simulink model "SimulationPPU_Simscape"  (R2026a)
settings: Solver=ode23t  StopTime=10  MaxStep=1e-6  RelTol=1e-4
InitFcn:
  | % Read the SETTINGS constants on the top level
  | ppu_mdl = bdroot; ppu_mws = get_param(ppu_mdl, 'ModelWorkspace');
  | ppu_Fsw = slResolve(get_param([ppu_mdl '/Switching frequency'], 'Value'), ppu_mdl);
  | ppu_Vb  = slResolve(get_param([ppu_mdl '/DC bus voltage'], 'Value'), ppu_mdl);
  | assignin(ppu_mws, 'V_bus', ppu_Vb);            % initial DC-link voltage
  | set_param(ppu_mdl, 'MaxStep', sprintf('%.6g', 1/(20*ppu_Fsw)));
  | clear ppu_mdl ppu_mws ppu_Fsw ppu_Vb
model workspace (MAT data in the model file):
  C_cer = 3.36e-06
  C_elec = 0.0033
  C_f = 0.00088
  C_film = 4.5e-05
  ESR_cer = 0.0008
  ESR_elec = 0.023
  ESR_f = 0.057
  ESR_film = 0.0011
  Ki_I = 0.7
  Kp = 50
  Kp_I = 0.008
  L_Rser = 0.001
  L_f = 5.3e-05
  L_load = 0.0059
  N_par = 4
  R_Vsrc = 0.1
  R_load = 0.5
  Rb = 0.012
  Rd = 0.0092
  Rds_eq = 0.00440383953356
  Rg_ext = 1
  Rgs = 10000
  Ron_diode = 0.003
  Rs = 0.0069
  T_log = 2e-06
  T_stop = 0.2
  V_bus = 400
  Vf_diode = 0.65
  Vgs_on = 17.99820018
  Vhigh = 18
  Vto = 4.8
  m_max = 1.15470053838
  tau_Imeas = 0.001
libraries: fl_lib x23, nesl_utility x19, ee_lib x6, slpidlib x1, simulink x1
(part 1 of 2)
settings Model: SimulationMode=accelerator  Creator=gonzalo  LastModifiedBy=gonzalo
settings SolverCC: InitialStep=1e-9  MaxConsecutiveZCs=100000  MaxConsecutiveMinStep=100000  ZeroCrossAlgorithm=Adaptive
settings DebuggingCC: MaxConsecutiveZCsMsg=none  MaskedZcDiagnostic=none  IgnoredZcDiagnostic=none

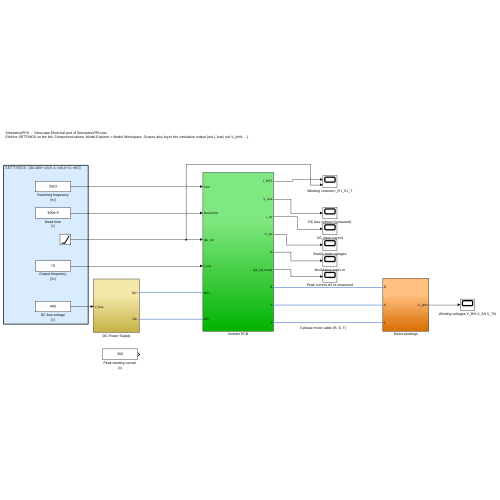
[thumbnail: Simulink's stored preview of the top-level diagram]
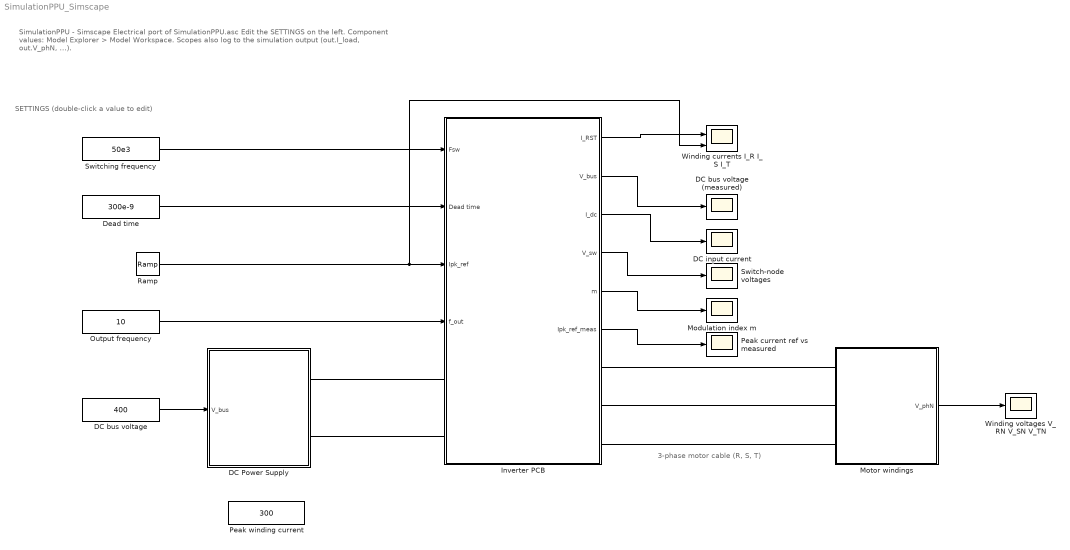
== system SimulationPPU_Simscape ==
  note: 3-phase motor cable (R, S, T)
  note: SETTINGS (double-click a value to edit)
  note: SimulationPPU  -  Simscape Electrical port of SimulationPPU.asc
      | Edit the SETTINGS on the left. Component values: Model Explorer > Model Workspace. Scopes also log to the simulation output (out.I_load, out.V_phN, ...).
  DC Power Supply : Subsystem
  DC bus voltage : Constant  Value=400
      settings: AttributesFormatString=[V]
  DC bus voltage (measured) : Scope
      settings: SampleTime=T_log  DataLoggingVariableName=V_bus_meas
  DC input current : Scope
      settings: SampleTime=T_log  DataLoggingVariableName=I_dc
  Dead time : Constant  Value=300e-9
      settings: AttributesFormatString=[s]
  Inverter PCB : Subsystem
  Modulation index m : Scope
      settings: SampleTime=T_log  DataLoggingVariableName=m
  Motor windings : Subsystem
  Output frequency : Constant  Value=10
      settings: AttributesFormatString=[Hz]
  Peak current ref vs measured : Scope
      settings: SampleTime=T_log  DataLoggingVariableName=Ipk_ref_meas
  Peak winding current : Constant  Value=300
      settings: AttributesFormatString=[A]
  Ramp : simulink/Sources/Ramp  slope=1  start=0  InitialOutput=10
  Switch-node voltages : Scope
      settings: SampleTime=T_log  DataLoggingVariableName=V_sw
  Switching frequency : Constant  Value=50e3
      settings: AttributesFormatString=[Hz]
  Winding currents I_R I_S I_T : Scope  NumInputPorts=2
      settings: SampleTime=T_log  DataLoggingVariableName=I_load
  Winding voltages V_RN V_SN V_TN : Scope
      settings: SampleTime=T_log  DataLoggingVariableName=V_phN
  wires:
  Switching frequency/1 -> Inverter PCB/1(Fsw)
  Dead time/1 -> Inverter PCB/2(Dead time)
  Ramp/1 -> Winding currents I_R I_S I_T/2, Inverter PCB/3(Ipk_ref)
  Output frequency/1 -> Inverter PCB/4(f_out)
  DC bus voltage/1 -> DC Power Supply/1(V_bus)
  Inverter PCB/1(I_RST) -> Winding currents I_R I_S I_T/1
  Inverter PCB/2(V_bus) -> DC bus voltage (measured)/1
  Inverter PCB/3(I_dc) -> DC input current/1
  Inverter PCB/4(V_sw) -> Switch-node voltages/1
  Inverter PCB/5(m) -> Modulation index m/1
  Inverter PCB/6(Ipk_ref_meas) -> Peak current ref vs measured/1
  Motor windings/1(V_phN) -> Winding voltages V_RN V_SN V_TN/1
  connections:
  DC Power Supply/RConn1 -- Inverter PCB/LConn1
  DC Power Supply/RConn2 -- Inverter PCB/LConn2
  Inverter PCB/RConn1 -- Motor windings/LConn1
  Inverter PCB/RConn2 -- Motor windings/LConn2
  Inverter PCB/RConn3 -- Motor windings/LConn3

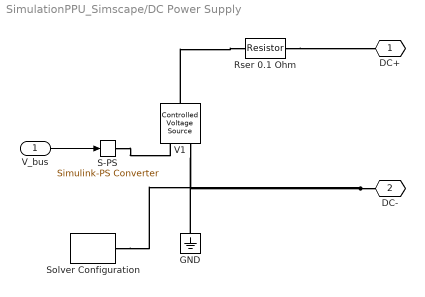
== system SimulationPPU_Simscape/DC Power Supply ==
  V_bus : Inport
  GND : fl_lib/Electrical/Electrical Elements/Electrical Reference
  Rser 0.1 Ohm : fl_lib/Electrical/Electrical Elements/Resistor  R=R_Vsrc Ohm  i_specify=off  i_priority=None  i=0 A  i_nominal_specify=off  i_nominal_value=1  i_nominal_unit=A  v_specify=off  v_priority=None  v=0 V  v_nominal_specify=off  v_nominal_value=1  v_nominal_unit=V
  S-PS : nesl_utility/Simulink-PS Converter  PhysicalDomain=network_engine_domain  SubClassName=ps_input  LeftPortType=input  RightPortType=output  PseudoPeriodic=off  Frequencies=[]  NoiseDistribution=none  NoiseParameters=[]  Unit=V  AffineConversion=off  FilteringAndDerivatives=zero  SimscapeFilterOrder=1  InputFilterTimeConstant=0.001  UdotUserProvided=0
  Solver Configuration : nesl_utility/Solver Configuration  PhysicalDomain=network_engine_domain  SubClassName=solver  LeftPortType=input  RightPortType=generic  Tones=[]  Harmonics=[]  SimulateNoise=off  Profile=off  UseLocalSampling=off  EnableSwitchedLinearOptims=on  FrequencyDomain=off  UseCCode=off  RelTol=0.001  AbsTol=0.001  MinStep=1e-09  ToWorkspace=off  RevertToSquareIcSolve=off  NumHomotopyIterations=100  PhasorMode=off  PhasorModeNumHarmonics=1  ConsistencySolver=NEWTON_XTOL_AFTER_FTOL  CanonicalOrdering=CANONICAL  OptimizeIntermediates=OPTIMIZED  IndexReductionMethod=DerivativeReplacement  DoDC=off  ResidualTolerance=1e-09  ConsistencyTolSource=GLOBAL  ConsistencyAbsTol=0.001  ConsistencyRelTol=0.001  ConsistencyTolFactor=0.001  UseLocalSolver=off  LocalSolverChoice=NE_BACKWARD_EULER_ADVANCER  ResolveIndetEquations=on  FunctionEvalNumThread=1  LocalSolverSampleTime=0.001  DoFixedCost=off  MaxNonlinIter=3  MaxModeIter=2  ComputeImpulses=off  ImpulseIterations=2  LinearAlgebra=auto  LinearAlgebraNumThread=0  EquationFormulation=NE_TIME_EF  DelaysMemoryBudget=1024  AutomaticFiltering=on  FilteringTimeConstant=0.001  PartitionStorageMethod=AS_NEEDED  PartitionMemoryBudget=1024  PartitionMethod=ROBUST  MultibodyUseLocalSolver=off  MultibodyLocalSolverChoice=ODE1  MultibodyLocalSolverSampleTime=0.001
  V1 : fl_lib/Electrical/Electrical Sources/Controlled Voltage Source
  DC+ : PMIOPort  Side=Right
  DC- : PMIOPort  Port=2  Side=Right
  wires:
  V_bus/1 -> S-PS/1
  connections:
  S-PS/RConn1 -- V1/RConn1
  V1/LConn1 -- Rser 0.1 Ohm/LConn1
  Rser 0.1 Ohm/RConn1 -- DC+/RConn1
  DC-/RConn1 -- V1/RConn2 -- GND/LConn1 -- Solver Configuration/RConn1

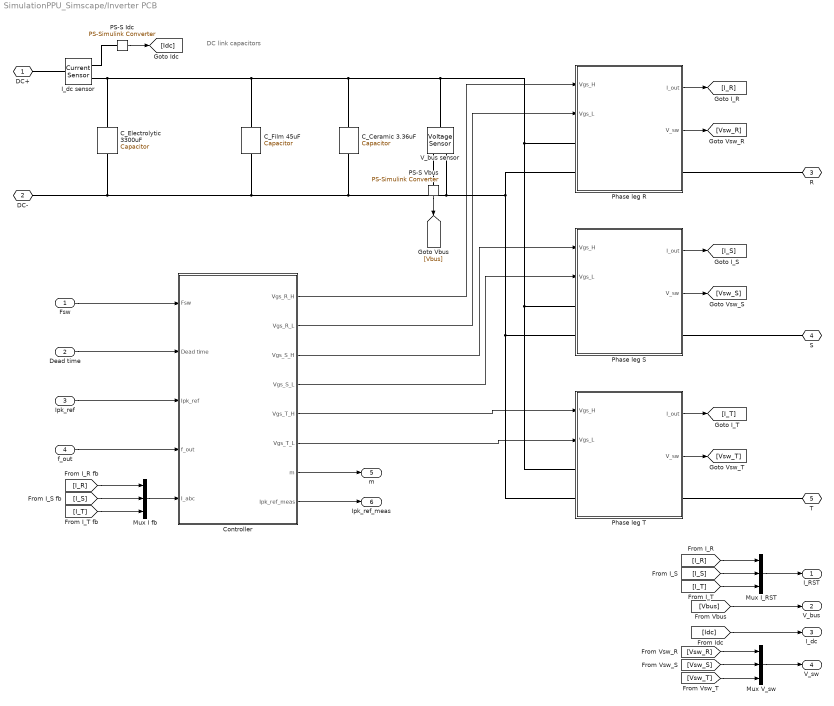
== system SimulationPPU_Simscape/Inverter PCB ==
  note: DC link capacitors
  Fsw : Inport
  Dead time : Inport  Port=2
  Ipk_ref : Inport  Port=3
  f_out : Inport  Port=4
  C_Ceramic 3.36uF : fl_lib/Electrical/Electrical Elements/Capacitor  c=C_cer F  r=ESR_cer Ohm  g=0 1/Ohm  i_specify=off  i_priority=None  i=0 A  i_nominal_specify=off  i_nominal_value=1  i_nominal_unit=A  v_specify=off  v_priority=None  v=0 V  v_nominal_specify=off  v_nominal_value=1  v_nominal_unit=V  vc_specify=on  vc_priority=High  vc=V_bus V  vc_nominal_specify=off  vc_nominal_value=1  vc_nominal_unit=V
  C_Electrolytic 3300uF : fl_lib/Electrical/Electrical Elements/Capacitor  c=C_elec F  r=ESR_elec Ohm  g=0 1/Ohm  i_specify=off  i_priority=None  i=0 A  i_nominal_specify=off  i_nominal_value=1  i_nominal_unit=A  v_specify=off  v_priority=None  v=0 V  v_nominal_specify=off  v_nominal_value=1  v_nominal_unit=V  vc_specify=on  vc_priority=High  vc=V_bus V  vc_nominal_specify=off  vc_nominal_value=1  vc_nominal_unit=V
  C_Film 45uF : fl_lib/Electrical/Electrical Elements/Capacitor  c=C_film F  r=ESR_film Ohm  g=0 1/Ohm  i_specify=off  i_priority=None  i=0 A  i_nominal_specify=off  i_nominal_value=1  i_nominal_unit=A  v_specify=off  v_priority=None  v=0 V  v_nominal_specify=off  v_nominal_value=1  v_nominal_unit=V  vc_specify=on  vc_priority=High  vc=V_bus V  vc_nominal_specify=off  vc_nominal_value=1  vc_nominal_unit=V
  Controller : Subsystem
  I_dc sensor : fl_lib/Electrical/Electrical Sensors/Current Sensor
  Mux I fb : Mux  Inputs=3
  Mux I_RST : Mux  Inputs=3
  Mux V_sw : Mux  Inputs=3
  PS-S Idc : nesl_utility/PS-Simulink Converter  PhysicalDomain=network_engine_domain  SubClassName=ps_output  LeftPortType=input  RightPortType=output  PseudoPeriodic=off  Frequencies=[]  VectorFormat=inherit  Unit=inherit  AffineConversion=off
  PS-S Vbus : nesl_utility/PS-Simulink Converter  PhysicalDomain=network_engine_domain  SubClassName=ps_output  LeftPortType=input  RightPortType=output  PseudoPeriodic=off  Frequencies=[]  VectorFormat=inherit  Unit=inherit  AffineConversion=off
  Phase leg R : Subsystem
  Phase leg S : Subsystem
  Phase leg T : Subsystem
  V_bus sensor : fl_lib/Electrical/Electrical Sensors/Voltage Sensor
  DC+ : PMIOPort  Side=Left
  DC- : PMIOPort  Port=2  Side=Left
  R : PMIOPort  Port=3  Side=Right
  S : PMIOPort  Port=4  Side=Right
  T : PMIOPort  Port=5  Side=Right
  I_RST : Outport
  V_bus : Outport  Port=2
  I_dc : Outport  Port=3
  V_sw : Outport  Port=4
  m : Outport  Port=5
  Ipk_ref_meas : Outport  Port=6
  wires:
  PS-S Idc/1 -> [Idc]
  PS-S Vbus/1 -> [Vbus]
  Phase leg R/1(I_out) -> [I_R]
  Phase leg R/2(V_sw) -> [Vsw_R]
  Phase leg S/1(I_out) -> [I_S]
  Phase leg S/2(V_sw) -> [Vsw_S]
  Phase leg T/1(I_out) -> [I_T]
  Phase leg T/2(V_sw) -> [Vsw_T]
  Fsw/1 -> Controller/1(Fsw)
  Dead time/1 -> Controller/2(Dead time)
  Ipk_ref/1 -> Controller/3(Ipk_ref)
  f_out/1 -> Controller/4(f_out)
  Mux I fb/1 -> Controller/5(I_abc)
  [I_R] -> Mux I fb/1
  [I_S] -> Mux I fb/2
  [I_T] -> Mux I fb/3
  Controller/1(Vgs_R_H) -> Phase leg R/1(Vgs_H)
  Controller/2(Vgs_R_L) -> Phase leg R/2(Vgs_L)
  Controller/3(Vgs_S_H) -> Phase leg S/1(Vgs_H)
  Controller/4(Vgs_S_L) -> Phase leg S/2(Vgs_L)
  Controller/5(Vgs_T_H) -> Phase leg T/1(Vgs_H)
  Controller/6(Vgs_T_L) -> Phase leg T/2(Vgs_L)
  Mux I_RST/1 -> I_RST/1
  [I_R] -> Mux I_RST/1
  [I_S] -> Mux I_RST/2
  [I_T] -> Mux I_RST/3
  Mux V_sw/1 -> V_sw/1
  [Vsw_R] -> Mux V_sw/1
  [Vsw_S] -> Mux V_sw/2
  [Vsw_T] -> Mux V_sw/3
  [Vbus] -> V_bus/1
  [Idc] -> I_dc/1
  Controller/7(m) -> m/1
  Controller/8(Ipk_ref_meas) -> Ipk_ref_meas/1
  connections:
  DC+/RConn1 -- I_dc sensor/LConn1
  I_dc sensor/RConn1 -- PS-S Idc/LConn1
  I_dc sensor/RConn2 -- C_Electrolytic 3300uF/LConn1 -- C_Film 45uF/LConn1 -- C_Ceramic 3.36uF/LConn1 -- V_bus sensor/LConn1 -- Phase leg R/LConn1 -- Phase leg S/LConn1 -- Phase leg T/LConn1
  DC-/RConn1 -- C_Electrolytic 3300uF/RConn1 -- C_Film 45uF/RConn1 -- C_Ceramic 3.36uF/RConn1 -- V_bus sensor/RConn2 -- Phase leg R/LConn2 -- Phase leg S/LConn2 -- Phase leg T/LConn2
  V_bus sensor/RConn1 -- PS-S Vbus/LConn1
  Phase leg R/RConn1 -- R/RConn1
  Phase leg S/RConn1 -- S/RConn1
  Phase leg T/RConn1 -- T/RConn1

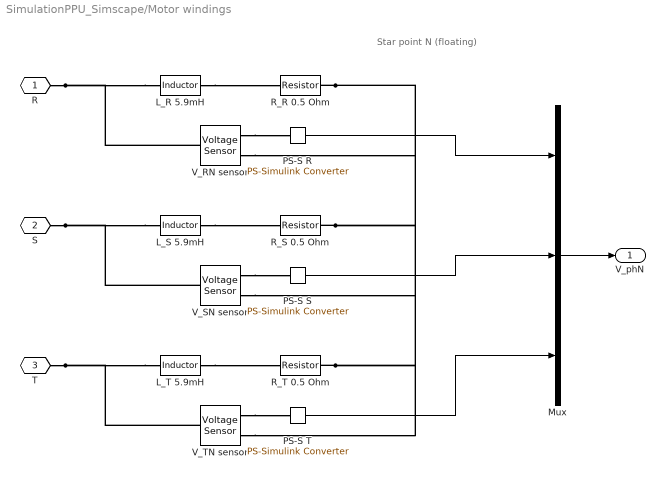
== system SimulationPPU_Simscape/Motor windings ==
  note: Star point N (floating)
  L_R 5.9mH : fl_lib/Electrical/Electrical Elements/Inductor  l=L_load H  r=L_Rser Ohm  g=0 1/Ohm  i_specify=off  i_priority=None  i=0 A  i_nominal_specify=off  i_nominal_value=1  i_nominal_unit=A  v_specify=off  v_priority=None  v=0 V  v_nominal_specify=off  v_nominal_value=1  v_nominal_unit=V  i_L_specify=off  i_L_priority=High  i_L=0 A  i_L_nominal_specify=off  i_L_nominal_value=1  i_L_nominal_unit=A
  L_S 5.9mH : fl_lib/Electrical/Electrical Elements/Inductor  l=L_load H  r=L_Rser Ohm  g=0 1/Ohm  i_specify=off  i_priority=None  i=0 A  i_nominal_specify=off  i_nominal_value=1  i_nominal_unit=A  v_specify=off  v_priority=None  v=0 V  v_nominal_specify=off  v_nominal_value=1  v_nominal_unit=V  i_L_specify=off  i_L_priority=High  i_L=0 A  i_L_nominal_specify=off  i_L_nominal_value=1  i_L_nominal_unit=A
  L_T 5.9mH : fl_lib/Electrical/Electrical Elements/Inductor  l=L_load H  r=L_Rser Ohm  g=0 1/Ohm  i_specify=off  i_priority=None  i=0 A  i_nominal_specify=off  i_nominal_value=1  i_nominal_unit=A  v_specify=off  v_priority=None  v=0 V  v_nominal_specify=off  v_nominal_value=1  v_nominal_unit=V  i_L_specify=off  i_L_priority=High  i_L=0 A  i_L_nominal_specify=off  i_L_nominal_value=1  i_L_nominal_unit=A
  Mux : Mux  Inputs=3
  PS-S R : nesl_utility/PS-Simulink Converter  PhysicalDomain=network_engine_domain  SubClassName=ps_output  LeftPortType=input  RightPortType=output  PseudoPeriodic=off  Frequencies=[]  VectorFormat=inherit  Unit=inherit  AffineConversion=off
  PS-S S : nesl_utility/PS-Simulink Converter  PhysicalDomain=network_engine_domain  SubClassName=ps_output  LeftPortType=input  RightPortType=output  PseudoPeriodic=off  Frequencies=[]  VectorFormat=inherit  Unit=inherit  AffineConversion=off
  PS-S T : nesl_utility/PS-Simulink Converter  PhysicalDomain=network_engine_domain  SubClassName=ps_output  LeftPortType=input  RightPortType=output  PseudoPeriodic=off  Frequencies=[]  VectorFormat=inherit  Unit=inherit  AffineConversion=off
  R_R 0.5 Ohm : fl_lib/Electrical/Electrical Elements/Resistor  R=R_load Ohm  i_specify=off  i_priority=None  i=0 A  i_nominal_specify=off  i_nominal_value=1  i_nominal_unit=A  v_specify=off  v_priority=None  v=0 V  v_nominal_specify=off  v_nominal_value=1  v_nominal_unit=V
  R_S 0.5 Ohm : fl_lib/Electrical/Electrical Elements/Resistor  R=R_load Ohm  i_specify=off  i_priority=None  i=0 A  i_nominal_specify=off  i_nominal_value=1  i_nominal_unit=A  v_specify=off  v_priority=None  v=0 V  v_nominal_specify=off  v_nominal_value=1  v_nominal_unit=V
  R_T 0.5 Ohm : fl_lib/Electrical/Electrical Elements/Resistor  R=R_load Ohm  i_specify=off  i_priority=None  i=0 A  i_nominal_specify=off  i_nominal_value=1  i_nominal_unit=A  v_specify=off  v_priority=None  v=0 V  v_nominal_specify=off  v_nominal_value=1  v_nominal_unit=V
  V_RN sensor : fl_lib/Electrical/Electrical Sensors/Voltage Sensor
  V_SN sensor : fl_lib/Electrical/Electrical Sensors/Voltage Sensor
  V_TN sensor : fl_lib/Electrical/Electrical Sensors/Voltage Sensor
  R : PMIOPort  Side=Left
  S : PMIOPort  Port=2  Side=Left
  T : PMIOPort  Port=3  Side=Left
  V_phN : Outport
  wires:
  Mux/1 -> V_phN/1
  PS-S R/1 -> Mux/1
  PS-S S/1 -> Mux/2
  PS-S T/1 -> Mux/3
  connections:
  L_R 5.9mH/LConn1 -- R/RConn1 -- V_RN sensor/LConn1
  L_R 5.9mH/RConn1 -- R_R 0.5 Ohm/LConn1
  R_R 0.5 Ohm/RConn1 -- V_RN sensor/RConn2 -- V_SN sensor/RConn2 -- R_S 0.5 Ohm/RConn1 -- V_TN sensor/RConn2 -- R_T 0.5 Ohm/RConn1
  V_RN sensor/RConn1 -- PS-S R/LConn1
  L_S 5.9mH/LConn1 -- S/RConn1 -- V_SN sensor/LConn1
  L_S 5.9mH/RConn1 -- R_S 0.5 Ohm/LConn1
  V_SN sensor/RConn1 -- PS-S S/LConn1
  L_T 5.9mH/LConn1 -- T/RConn1 -- V_TN sensor/LConn1
  L_T 5.9mH/RConn1 -- R_T 0.5 Ohm/LConn1
  V_TN sensor/RConn1 -- PS-S T/LConn1

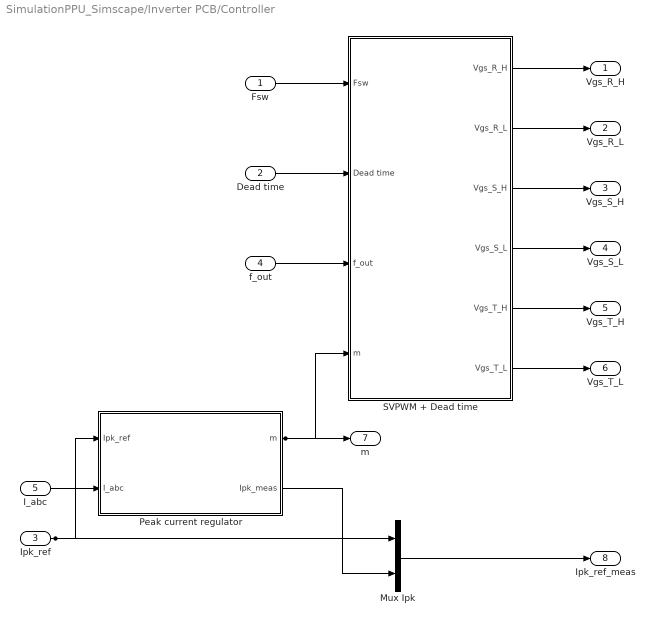
== system SimulationPPU_Simscape/Inverter PCB/Controller ==
  Fsw : Inport
  Dead time : Inport  Port=2
  Ipk_ref : Inport  Port=3
  f_out : Inport  Port=4
  I_abc : Inport  Port=5
  Mux Ipk : Mux  Inputs=2
  Peak current regulator : Subsystem
  SVPWM + Dead time : Subsystem
  Vgs_R_H : Outport
  Vgs_R_L : Outport  Port=2
  Vgs_S_H : Outport  Port=3
  Vgs_S_L : Outport  Port=4
  Vgs_T_H : Outport  Port=5
  Vgs_T_L : Outport  Port=6
  m : Outport  Port=7
  Ipk_ref_meas : Outport  Port=8
  wires:
  Mux Ipk/1 -> Ipk_ref_meas/1
  I_abc/1 -> Peak current regulator/2(I_abc)
  Peak current regulator/1(m) -> m/1, SVPWM + Dead time/4(m)
  Ipk_ref/1 -> Peak current regulator/1(Ipk_ref), Mux Ipk/1
  SVPWM + Dead time/5(Vgs_T_H) -> Vgs_T_H/1
  Fsw/1 -> SVPWM + Dead time/1(Fsw)
  SVPWM + Dead time/4(Vgs_S_L) -> Vgs_S_L/1
  Dead time/1 -> SVPWM + Dead time/2(Dead time)
  SVPWM + Dead time/2(Vgs_R_L) -> Vgs_R_L/1
  f_out/1 -> SVPWM + Dead time/3(f_out)
  SVPWM + Dead time/1(Vgs_R_H) -> Vgs_R_H/1
  Peak current regulator/2(Ipk_meas) -> Mux Ipk/2
  SVPWM + Dead time/6(Vgs_T_L) -> Vgs_T_L/1
  SVPWM + Dead time/3(Vgs_S_H) -> Vgs_S_H/1

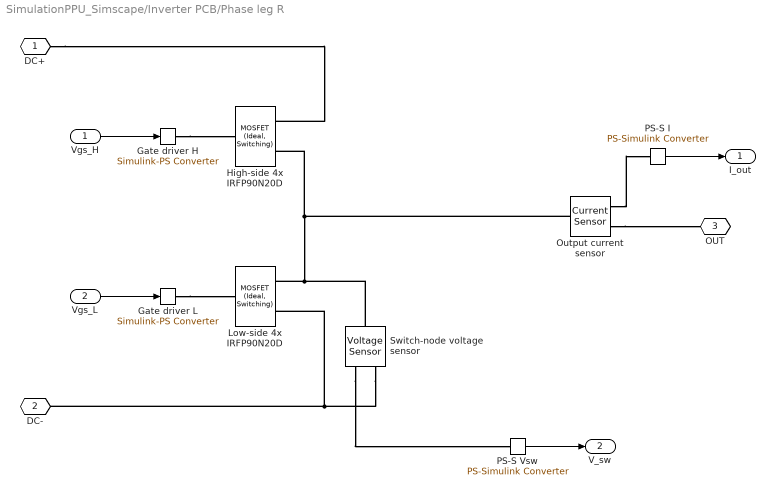
== system SimulationPPU_Simscape/Inverter PCB/Phase leg R ==
  Vgs_H : Inport
  Vgs_L : Inport  Port=2
  Gate driver H : nesl_utility/Simulink-PS Converter  PhysicalDomain=network_engine_domain  SubClassName=ps_input  LeftPortType=input  RightPortType=output  PseudoPeriodic=off  Frequencies=[]  NoiseDistribution=none  NoiseParameters=[]  Unit=V  AffineConversion=off  FilteringAndDerivatives=zero  SimscapeFilterOrder=1  InputFilterTimeConstant=0.001  UdotUserProvided=0
  Gate driver L : nesl_utility/Simulink-PS Converter  PhysicalDomain=network_engine_domain  SubClassName=ps_input  LeftPortType=input  RightPortType=output  PseudoPeriodic=off  Frequencies=[]  NoiseDistribution=none  NoiseParameters=[]  Unit=V  AffineConversion=off  FilteringAndDerivatives=zero  SimscapeFilterOrder=1  InputFilterTimeConstant=0.001  UdotUserProvided=0
  High-side 4x IRFP90N20D : ee_lib/Semiconductors & Converters/MOSFET (Ideal, Switching)  port_option=ee.enum.controlport.ps  Rds=Rds_eq Ohm  Goff=1e-7 1/Ohm  Vth=Vto V  diode_param=ee.enum.semiconductors.protectionDiode.nodynamics  diode_Vf=Vf_diode V  diode_Ron=Ron_diode Ohm  diode_Goff=1e-7 1/Ohm  diode_C=50e-9 F  diode_iRM=-235 A  diode_iF=300 A  diode_idot=-50 A/us  diode_trr_param=ee.enum.converters.diodeReverseParam.trr_factor  diode_trr_factor=3  diode_trr=15 us  diode_Qrr=1500 s*uA  ids_specify=off  ids_priority=None  ids=0 A  ids_nominal_specify=off  ids_nominal_value=1  ids_nominal_unit=A  vds_specify=off  vds_priority=None  vds=0 V  vds_nominal_specify=off  vds_nominal_value=1  vds_nominal_unit=V  vgs_specify=off  vgs_priority=None  vgs=0 V  vgs_nominal_specify=off  vgs_nominal_value=1  vgs_nominal_unit=V  thermal_loss_option=ee.enum.converters.thermalLossOption.constantvalues  Von_data=[0, 1.8, 3.2, 6, 10, 16; 0, 2, 5.5, 9.5, 15, 25] V  Tj=[298.15, 448.15] K  Iout_data=[0, 20, 40, 60, 80, 100] A  tabulateWithVds=false  Eon_data=[0, 55.04, 124.57, 235.53, 362.12; 0, 71.25, 161.25, 304.88, 468.75] * 1e-6 J  Eoff_data=[0, 18, 30, 56.1, 76.5; 0, 22.5, 37.5, 70.13, 95.63] * 1e-6 J  Eon_data_3D=[zeros(2, 5, 3)] J  Eoff_data_3D=[zeros(2, 5, 3)] J  Tj_loss=[298.15, 448.15] K  Iout_data_loss=[0, 10, 20, 30, 40] A  Vds_loss=[0, 150, 300] V  Eon_scalar=22.86e-3 J  Eoff_scalar=17.14e-3 J  Voff=300 V  Iout_scalar=600 A  useCurrentFromPreviousCycle=false  useVoltageFromPreviousCycle=false  diodeModelType=ee.enum.converters.diodeModelType.pwl  diodeTableType=ee.enum.diode.tableType.IfMat  diode_ReverseIVType=ee.enum.diode.diodeReverseIV.constant  diode_IfMat=[.07, .12, .19, 1.75, 4.24, 7.32, 11.2; .16, .3, .72, 2.14, 4.02, 6.35, 9.12] A  diode_VfMat=[.9, 1.15, 1.25, 1.5, 1.75, 2.17, 2.6, 2.85; .58, .68, .75, 1.1, 1.38, 1.77, 2.27, 2.7] V  diode_TjVec=[25, 125] degC  diode_VfVec=[.5, .7, .9, 1.3, 1.7, 2.1, 2.5] V  diode_IfVec=[.1, .2, .5, 1, 2, 4, 7, 10] A  diode_IrMat=[1e-06, 2e-06, 5e-06, 1e-05, 2.5e-05, 5e-05, .0001; 2e-06, 5e-06, 1e-05, 4e-05, 8e-05, .0002, .0005] A  diode_VrMat=[10, 100, 200, 250, 300, 325, 350; 10, 70, 160, 220, 270, 300, 320] V  diode_VrVec=[10, 20, 40, 50, 70, 80, 100] V  diode_IrVec=[1e-06, 2e-06, 5e-06, 1e-05, 2e-05, 5e-05, .0001] A  diode_Vr=-600 V  diode_Ls=150 nH  diode_Erec=0.03 J  diode_rec_loss_model=ee.enum.diode.reverseRecoveryModelTabulateUpTo3D.fixed  diode_ErecVal=0 J  diode_scaleWithIandV=true  diode_ErecMat=zeros(2, 3) J  diodeErecMat3D=zeros(2, 3, 2) J  diode_TjrecVec=[298.15, 398.15] K  diode_IfrecVec=[.1, 1, 10] A  diodeVrecVec=[0, 100] V  diode_IrecVal=10 A  diode_VrecVal=10 V  diode_tFilter=1 / 1000 / 100 s  separateThermalPortForDiode=false  thermal_network_parameterization=ee.enum.thermalNetworkTopology.external  Rth=[.03, .2] K/W  Rth_Cauer=[.03, .1, .2] K/W  Rth_Foster=[.08, .14, .22, .16] K/W  thermal_mass_parameterization=ee.enum.thermalNetwork.timeconstant  thermal_mass=[3, 25] J/K  thermal_mass_Cauer=[3, 10, 25] J/K  thermal_mass_Foster=[.001, .005, .05, .5] J/K  thermal_time_constant=[.1, 5] s  thermal_time_constant_Cauer=[.1, 1, 5] s  thermal_time_constant_Foster=[7e-05, .0007, .01, .08] s  thermal_mass_initial_temperatures=[25, 25] degC  thermal_mass_initial_temperatures_Cauer=[25, 25, 25] degC  junction_thermal_mass=0.1 J/K  Tvec_initial_Foster=[25, 25, 25, 25] degC  RthDiode=[.03, .2] K/W  RthCauerDiode=[.03, .1, .2] K/W  RthFosterDiode=[.03, .2] K/W  thermalMassDiode=[3, 25] J/K  thermalMassCauerDiode=[3, 10, 25] J/K  thermalMassFosterDiode=[33, 50] J/K  thermalTauDiode=[.1, 5] s  thermalTauCauerDiode=[.1, 1, 5] s  thermalTauFosterDiode=[1, 10] s  thermalMassInitTempDiode=[25, 25] degC  thermalMassInitTempCauerDiode=[25, 25, 25] degC  junctionthermalMassDiode=0.1 J/K  TVecInitialFosterDiode=[25, 25, 25, 25] degC  no_thermal_network=ee.enum.enable.no  mosfet_junction_temperature_specify=off  mosfet_junction_temperature_priority=None  mosfet_junction_temperature=25 degC  mosfet_junction_temperature_nominal_specify=off  mosfet_junction_temperature_nominal_value=1  mosfet_junction_temperature_nominal_unit=degC  diode_junction_temperature_specify=off  diode_junction_temperature_priority=None  diode_junction_temperature=25 degC  diode_junction_temperature_nominal_specify=off  diode_junction_temperature_nominal_value=1  diode_junction_temperature_nominal_unit=degC  Qj_specify=off  Qj_priority=None  Qj=0 W  Qj_nominal_specify=off  Qj_nominal_value=1  Qj_nominal_unit=W  accumulatedSwitchingLosses_specify=off  accumulatedSwitchingLosses_priority=None  accumulatedSwitchingLosses=0 J
  Low-side 4x IRFP90N20D : ee_lib/Semiconductors & Converters/MOSFET (Ideal, Switching)  port_option=ee.enum.controlport.ps  Rds=Rds_eq Ohm  Goff=1e-7 1/Ohm  Vth=Vto V  diode_param=ee.enum.semiconductors.protectionDiode.nodynamics  diode_Vf=Vf_diode V  diode_Ron=Ron_diode Ohm  diode_Goff=1e-7 1/Ohm  diode_C=50e-9 F  diode_iRM=-235 A  diode_iF=300 A  diode_idot=-50 A/us  diode_trr_param=ee.enum.converters.diodeReverseParam.trr_factor  diode_trr_factor=3  diode_trr=15 us  diode_Qrr=1500 s*uA  ids_specify=off  ids_priority=None  ids=0 A  ids_nominal_specify=off  ids_nominal_value=1  ids_nominal_unit=A  vds_specify=off  vds_priority=None  vds=0 V  vds_nominal_specify=off  vds_nominal_value=1  vds_nominal_unit=V  vgs_specify=off  vgs_priority=None  vgs=0 V  vgs_nominal_specify=off  vgs_nominal_value=1  vgs_nominal_unit=V  thermal_loss_option=ee.enum.converters.thermalLossOption.constantvalues  Von_data=[0, 1.8, 3.2, 6, 10, 16; 0, 2, 5.5, 9.5, 15, 25] V  Tj=[298.15, 448.15] K  Iout_data=[0, 20, 40, 60, 80, 100] A  tabulateWithVds=false  Eon_data=[0, 55.04, 124.57, 235.53, 362.12; 0, 71.25, 161.25, 304.88, 468.75] * 1e-6 J  Eoff_data=[0, 18, 30, 56.1, 76.5; 0, 22.5, 37.5, 70.13, 95.63] * 1e-6 J  Eon_data_3D=[zeros(2, 5, 3)] J  Eoff_data_3D=[zeros(2, 5, 3)] J  Tj_loss=[298.15, 448.15] K  Iout_data_loss=[0, 10, 20, 30, 40] A  Vds_loss=[0, 150, 300] V  Eon_scalar=22.86e-3 J  Eoff_scalar=17.14e-3 J  Voff=300 V  Iout_scalar=600 A  useCurrentFromPreviousCycle=false  useVoltageFromPreviousCycle=false  diodeModelType=ee.enum.converters.diodeModelType.pwl  diodeTableType=ee.enum.diode.tableType.IfMat  diode_ReverseIVType=ee.enum.diode.diodeReverseIV.constant  diode_IfMat=[.07, .12, .19, 1.75, 4.24, 7.32, 11.2; .16, .3, .72, 2.14, 4.02, 6.35, 9.12] A  diode_VfMat=[.9, 1.15, 1.25, 1.5, 1.75, 2.17, 2.6, 2.85; .58, .68, .75, 1.1, 1.38, 1.77, 2.27, 2.7] V  diode_TjVec=[25, 125] degC  diode_VfVec=[.5, .7, .9, 1.3, 1.7, 2.1, 2.5] V  diode_IfVec=[.1, .2, .5, 1, 2, 4, 7, 10] A  diode_IrMat=[1e-06, 2e-06, 5e-06, 1e-05, 2.5e-05, 5e-05, .0001; 2e-06, 5e-06, 1e-05, 4e-05, 8e-05, .0002, .0005] A  diode_VrMat=[10, 100, 200, 250, 300, 325, 350; 10, 70, 160, 220, 270, 300, 320] V  diode_VrVec=[10, 20, 40, 50, 70, 80, 100] V  diode_IrVec=[1e-06, 2e-06, 5e-06, 1e-05, 2e-05, 5e-05, .0001] A  diode_Vr=-600 V  diode_Ls=150 nH  diode_Erec=0.03 J  diode_rec_loss_model=ee.enum.diode.reverseRecoveryModelTabulateUpTo3D.fixed  diode_ErecVal=0 J  diode_scaleWithIandV=true  diode_ErecMat=zeros(2, 3) J  diodeErecMat3D=zeros(2, 3, 2) J  diode_TjrecVec=[298.15, 398.15] K  diode_IfrecVec=[.1, 1, 10] A  diodeVrecVec=[0, 100] V  diode_IrecVal=10 A  diode_VrecVal=10 V  diode_tFilter=1 / 1000 / 100 s  separateThermalPortForDiode=false  thermal_network_parameterization=ee.enum.thermalNetworkTopology.external  Rth=[.03, .2] K/W  Rth_Cauer=[.03, .1, .2] K/W  Rth_Foster=[.08, .14, .22, .16] K/W  thermal_mass_parameterization=ee.enum.thermalNetwork.timeconstant  thermal_mass=[3, 25] J/K  thermal_mass_Cauer=[3, 10, 25] J/K  thermal_mass_Foster=[.001, .005, .05, .5] J/K  thermal_time_constant=[.1, 5] s  thermal_time_constant_Cauer=[.1, 1, 5] s  thermal_time_constant_Foster=[7e-05, .0007, .01, .08] s  thermal_mass_initial_temperatures=[25, 25] degC  thermal_mass_initial_temperatures_Cauer=[25, 25, 25] degC  junction_thermal_mass=0.1 J/K  Tvec_initial_Foster=[25, 25, 25, 25] degC  RthDiode=[.03, .2] K/W  RthCauerDiode=[.03, .1, .2] K/W  RthFosterDiode=[.03, .2] K/W  thermalMassDiode=[3, 25] J/K  thermalMassCauerDiode=[3, 10, 25] J/K  thermalMassFosterDiode=[33, 50] J/K  thermalTauDiode=[.1, 5] s  thermalTauCauerDiode=[.1, 1, 5] s  thermalTauFosterDiode=[1, 10] s  thermalMassInitTempDiode=[25, 25] degC  thermalMassInitTempCauerDiode=[25, 25, 25] degC  junctionthermalMassDiode=0.1 J/K  TVecInitialFosterDiode=[25, 25, 25, 25] degC  no_thermal_network=ee.enum.enable.no  mosfet_junction_temperature_specify=off  mosfet_junction_temperature_priority=None  mosfet_junction_temperature=25 degC  mosfet_junction_temperature_nominal_specify=off  mosfet_junction_temperature_nominal_value=1  mosfet_junction_temperature_nominal_unit=degC  diode_junction_temperature_specify=off  diode_junction_temperature_priority=None  diode_junction_temperature=25 degC  diode_junction_temperature_nominal_specify=off  diode_junction_temperature_nominal_value=1  diode_junction_temperature_nominal_unit=degC  Qj_specify=off  Qj_priority=None  Qj=0 W  Qj_nominal_specify=off  Qj_nominal_value=1  Qj_nominal_unit=W  accumulatedSwitchingLosses_specify=off  accumulatedSwitchingLosses_priority=None  accumulatedSwitchingLosses=0 J
  Output current sensor : fl_lib/Electrical/Electrical Sensors/Current Sensor
  PS-S I : nesl_utility/PS-Simulink Converter  PhysicalDomain=network_engine_domain  SubClassName=ps_output  LeftPortType=input  RightPortType=output  PseudoPeriodic=off  Frequencies=[]  VectorFormat=inherit  Unit=inherit  AffineConversion=off
  PS-S Vsw : nesl_utility/PS-Simulink Converter  PhysicalDomain=network_engine_domain  SubClassName=ps_output  LeftPortType=input  RightPortType=output  PseudoPeriodic=off  Frequencies=[]  VectorFormat=inherit  Unit=inherit  AffineConversion=off
  Switch-node voltage sensor : fl_lib/Electrical/Electrical Sensors/Voltage Sensor
  DC+ : PMIOPort  Side=Left
  DC- : PMIOPort  Port=2  Side=Left
  OUT : PMIOPort  Port=3  Side=Right
  I_out : Outport
  V_sw : Outport  Port=2
  wires:
  Vgs_H/1 -> Gate driver H/1
  Vgs_L/1 -> Gate driver L/1
  PS-S I/1 -> I_out/1
  PS-S Vsw/1 -> V_sw/1
  connections:
  Gate driver H/RConn1 -- High-side 4x IRFP90N20D/LConn1
  Gate driver L/RConn1 -- Low-side 4x IRFP90N20D/LConn1
  DC+/RConn1 -- High-side 4x IRFP90N20D/RConn1
  Output current sensor/LConn1 -- High-side 4x IRFP90N20D/RConn2 -- Low-side 4x IRFP90N20D/RConn1 -- Switch-node voltage sensor/LConn1
  DC-/RConn1 -- Switch-node voltage sensor/RConn2 -- Low-side 4x IRFP90N20D/RConn2
  Output current sensor/RConn2 -- OUT/RConn1
  Output current sensor/RConn1 -- PS-S I/LConn1
  Switch-node voltage sensor/RConn1 -- PS-S Vsw/LConn1

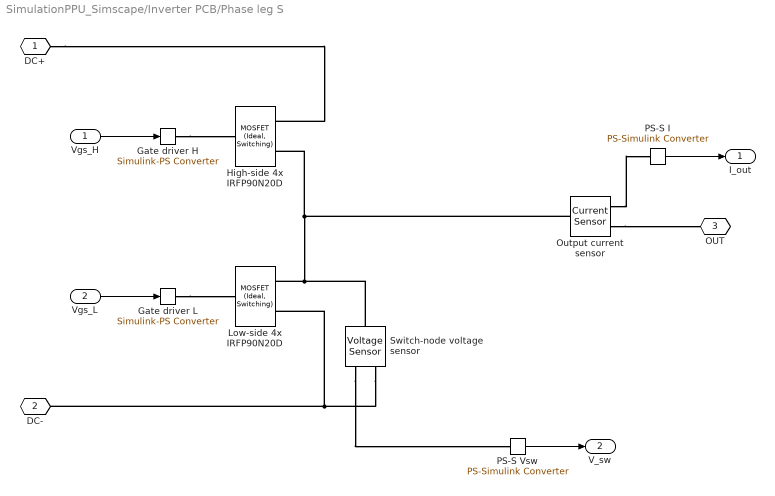
== system SimulationPPU_Simscape/Inverter PCB/Phase leg S ==
  Vgs_H : Inport
  Vgs_L : Inport  Port=2
  Gate driver H : nesl_utility/Simulink-PS Converter  PhysicalDomain=network_engine_domain  SubClassName=ps_input  LeftPortType=input  RightPortType=output  PseudoPeriodic=off  Frequencies=[]  NoiseDistribution=none  NoiseParameters=[]  Unit=V  AffineConversion=off  FilteringAndDerivatives=zero  SimscapeFilterOrder=1  InputFilterTimeConstant=0.001  UdotUserProvided=0
  Gate driver L : nesl_utility/Simulink-PS Converter  PhysicalDomain=network_engine_domain  SubClassName=ps_input  LeftPortType=input  RightPortType=output  PseudoPeriodic=off  Frequencies=[]  NoiseDistribution=none  NoiseParameters=[]  Unit=V  AffineConversion=off  FilteringAndDerivatives=zero  SimscapeFilterOrder=1  InputFilterTimeConstant=0.001  UdotUserProvided=0
  High-side 4x IRFP90N20D : ee_lib/Semiconductors & Converters/MOSFET (Ideal, Switching)  port_option=ee.enum.controlport.ps  Rds=Rds_eq Ohm  Goff=1e-7 1/Ohm  Vth=Vto V  diode_param=ee.enum.semiconductors.protectionDiode.nodynamics  diode_Vf=Vf_diode V  diode_Ron=Ron_diode Ohm  diode_Goff=1e-7 1/Ohm  diode_C=50e-9 F  diode_iRM=-235 A  diode_iF=300 A  diode_idot=-50 A/us  diode_trr_param=ee.enum.converters.diodeReverseParam.trr_factor  diode_trr_factor=3  diode_trr=15 us  diode_Qrr=1500 s*uA  ids_specify=off  ids_priority=None  ids=0 A  ids_nominal_specify=off  ids_nominal_value=1  ids_nominal_unit=A  vds_specify=off  vds_priority=None  vds=0 V  vds_nominal_specify=off  vds_nominal_value=1  vds_nominal_unit=V  vgs_specify=off  vgs_priority=None  vgs=0 V  vgs_nominal_specify=off  vgs_nominal_value=1  vgs_nominal_unit=V  thermal_loss_option=ee.enum.converters.thermalLossOption.constantvalues  Von_data=[0, 1.8, 3.2, 6, 10, 16; 0, 2, 5.5, 9.5, 15, 25] V  Tj=[298.15, 448.15] K  Iout_data=[0, 20, 40, 60, 80, 100] A  tabulateWithVds=false  Eon_data=[0, 55.04, 124.57, 235.53, 362.12; 0, 71.25, 161.25, 304.88, 468.75] * 1e-6 J  Eoff_data=[0, 18, 30, 56.1, 76.5; 0, 22.5, 37.5, 70.13, 95.63] * 1e-6 J  Eon_data_3D=[zeros(2, 5, 3)] J  Eoff_data_3D=[zeros(2, 5, 3)] J  Tj_loss=[298.15, 448.15] K  Iout_data_loss=[0, 10, 20, 30, 40] A  Vds_loss=[0, 150, 300] V  Eon_scalar=22.86e-3 J  Eoff_scalar=17.14e-3 J  Voff=300 V  Iout_scalar=600 A  useCurrentFromPreviousCycle=false  useVoltageFromPreviousCycle=false  diodeModelType=ee.enum.converters.diodeModelType.pwl  diodeTableType=ee.enum.diode.tableType.IfMat  diode_ReverseIVType=ee.enum.diode.diodeReverseIV.constant  diode_IfMat=[.07, .12, .19, 1.75, 4.24, 7.32, 11.2; .16, .3, .72, 2.14, 4.02, 6.35, 9.12] A  diode_VfMat=[.9, 1.15, 1.25, 1.5, 1.75, 2.17, 2.6, 2.85; .58, .68, .75, 1.1, 1.38, 1.77, 2.27, 2.7] V  diode_TjVec=[25, 125] degC  diode_VfVec=[.5, .7, .9, 1.3, 1.7, 2.1, 2.5] V  diode_IfVec=[.1, .2, .5, 1, 2, 4, 7, 10] A  diode_IrMat=[1e-06, 2e-06, 5e-06, 1e-05, 2.5e-05, 5e-05, .0001; 2e-06, 5e-06, 1e-05, 4e-05, 8e-05, .0002, .0005] A  diode_VrMat=[10, 100, 200, 250, 300, 325, 350; 10, 70, 160, 220, 270, 300, 320] V  diode_VrVec=[10, 20, 40, 50, 70, 80, 100] V  diode_IrVec=[1e-06, 2e-06, 5e-06, 1e-05, 2e-05, 5e-05, .0001] A  diode_Vr=-600 V  diode_Ls=150 nH  diode_Erec=0.03 J  diode_rec_loss_model=ee.enum.diode.reverseRecoveryModelTabulateUpTo3D.fixed  diode_ErecVal=0 J  diode_scaleWithIandV=true  diode_ErecMat=zeros(2, 3) J  diodeErecMat3D=zeros(2, 3, 2) J  diode_TjrecVec=[298.15, 398.15] K  diode_IfrecVec=[.1, 1, 10] A  diodeVrecVec=[0, 100] V  diode_IrecVal=10 A  diode_VrecVal=10 V  diode_tFilter=1 / 1000 / 100 s  separateThermalPortForDiode=false  thermal_network_parameterization=ee.enum.thermalNetworkTopology.external  Rth=[.03, .2] K/W  Rth_Cauer=[.03, .1, .2] K/W  Rth_Foster=[.08, .14, .22, .16] K/W  thermal_mass_parameterization=ee.enum.thermalNetwork.timeconstant  thermal_mass=[3, 25] J/K  thermal_mass_Cauer=[3, 10, 25] J/K  thermal_mass_Foster=[.001, .005, .05, .5] J/K  thermal_time_constant=[.1, 5] s  thermal_time_constant_Cauer=[.1, 1, 5] s  thermal_time_constant_Foster=[7e-05, .0007, .01, .08] s  thermal_mass_initial_temperatures=[25, 25] degC  thermal_mass_initial_temperatures_Cauer=[25, 25, 25] degC  junction_thermal_mass=0.1 J/K  Tvec_initial_Foster=[25, 25, 25, 25] degC  RthDiode=[.03, .2] K/W  RthCauerDiode=[.03, .1, .2] K/W  RthFosterDiode=[.03, .2] K/W  thermalMassDiode=[3, 25] J/K  thermalMassCauerDiode=[3, 10, 25] J/K  thermalMassFosterDiode=[33, 50] J/K  thermalTauDiode=[.1, 5] s  thermalTauCauerDiode=[.1, 1, 5] s  thermalTauFosterDiode=[1, 10] s  thermalMassInitTempDiode=[25, 25] degC  thermalMassInitTempCauerDiode=[25, 25, 25] degC  junctionthermalMassDiode=0.1 J/K  TVecInitialFosterDiode=[25, 25, 25, 25] degC  no_thermal_network=ee.enum.enable.no  mosfet_junction_temperature_specify=off  mosfet_junction_temperature_priority=None  mosfet_junction_temperature=25 degC  mosfet_junction_temperature_nominal_specify=off  mosfet_junction_temperature_nominal_value=1  mosfet_junction_temperature_nominal_unit=degC  diode_junction_temperature_specify=off  diode_junction_temperature_priority=None  diode_junction_temperature=25 degC  diode_junction_temperature_nominal_specify=off  diode_junction_temperature_nominal_value=1  diode_junction_temperature_nominal_unit=degC  Qj_specify=off  Qj_priority=None  Qj=0 W  Qj_nominal_specify=off  Qj_nominal_value=1  Qj_nominal_unit=W  accumulatedSwitchingLosses_specify=off  accumulatedSwitchingLosses_priority=None  accumulatedSwitchingLosses=0 J
  Low-side 4x IRFP90N20D : ee_lib/Semiconductors & Converters/MOSFET (Ideal, Switching)  port_option=ee.enum.controlport.ps  Rds=Rds_eq Ohm  Goff=1e-7 1/Ohm  Vth=Vto V  diode_param=ee.enum.semiconductors.protectionDiode.nodynamics  diode_Vf=Vf_diode V  diode_Ron=Ron_diode Ohm  diode_Goff=1e-7 1/Ohm  diode_C=50e-9 F  diode_iRM=-235 A  diode_iF=300 A  diode_idot=-50 A/us  diode_trr_param=ee.enum.converters.diodeReverseParam.trr_factor  diode_trr_factor=3  diode_trr=15 us  diode_Qrr=1500 s*uA  ids_specify=off  ids_priority=None  ids=0 A  ids_nominal_specify=off  ids_nominal_value=1  ids_nominal_unit=A  vds_specify=off  vds_priority=None  vds=0 V  vds_nominal_specify=off  vds_nominal_value=1  vds_nominal_unit=V  vgs_specify=off  vgs_priority=None  vgs=0 V  vgs_nominal_specify=off  vgs_nominal_value=1  vgs_nominal_unit=V  thermal_loss_option=ee.enum.converters.thermalLossOption.constantvalues  Von_data=[0, 1.8, 3.2, 6, 10, 16; 0, 2, 5.5, 9.5, 15, 25] V  Tj=[298.15, 448.15] K  Iout_data=[0, 20, 40, 60, 80, 100] A  tabulateWithVds=false  Eon_data=[0, 55.04, 124.57, 235.53, 362.12; 0, 71.25, 161.25, 304.88, 468.75] * 1e-6 J  Eoff_data=[0, 18, 30, 56.1, 76.5; 0, 22.5, 37.5, 70.13, 95.63] * 1e-6 J  Eon_data_3D=[zeros(2, 5, 3)] J  Eoff_data_3D=[zeros(2, 5, 3)] J  Tj_loss=[298.15, 448.15] K  Iout_data_loss=[0, 10, 20, 30, 40] A  Vds_loss=[0, 150, 300] V  Eon_scalar=22.86e-3 J  Eoff_scalar=17.14e-3 J  Voff=300 V  Iout_scalar=600 A  useCurrentFromPreviousCycle=false  useVoltageFromPreviousCycle=false  diodeModelType=ee.enum.converters.diodeModelType.pwl  diodeTableType=ee.enum.diode.tableType.IfMat  diode_ReverseIVType=ee.enum.diode.diodeReverseIV.constant  diode_IfMat=[.07, .12, .19, 1.75, 4.24, 7.32, 11.2; .16, .3, .72, 2.14, 4.02, 6.35, 9.12] A  diode_VfMat=[.9, 1.15, 1.25, 1.5, 1.75, 2.17, 2.6, 2.85; .58, .68, .75, 1.1, 1.38, 1.77, 2.27, 2.7] V  diode_TjVec=[25, 125] degC  diode_VfVec=[.5, .7, .9, 1.3, 1.7, 2.1, 2.5] V  diode_IfVec=[.1, .2, .5, 1, 2, 4, 7, 10] A  diode_IrMat=[1e-06, 2e-06, 5e-06, 1e-05, 2.5e-05, 5e-05, .0001; 2e-06, 5e-06, 1e-05, 4e-05, 8e-05, .0002, .0005] A  diode_VrMat=[10, 100, 200, 250, 300, 325, 350; 10, 70, 160, 220, 270, 300, 320] V  diode_VrVec=[10, 20, 40, 50, 70, 80, 100] V  diode_IrVec=[1e-06, 2e-06, 5e-06, 1e-05, 2e-05, 5e-05, .0001] A  diode_Vr=-600 V  diode_Ls=150 nH  diode_Erec=0.03 J  diode_rec_loss_model=ee.enum.diode.reverseRecoveryModelTabulateUpTo3D.fixed  diode_ErecVal=0 J  diode_scaleWithIandV=true  diode_ErecMat=zeros(2, 3) J  diodeErecMat3D=zeros(2, 3, 2) J  diode_TjrecVec=[298.15, 398.15] K  diode_IfrecVec=[.1, 1, 10] A  diodeVrecVec=[0, 100] V  diode_IrecVal=10 A  diode_VrecVal=10 V  diode_tFilter=1 / 1000 / 100 s  separateThermalPortForDiode=false  thermal_network_parameterization=ee.enum.thermalNetworkTopology.external  Rth=[.03, .2] K/W  Rth_Cauer=[.03, .1, .2] K/W  Rth_Foster=[.08, .14, .22, .16] K/W  thermal_mass_parameterization=ee.enum.thermalNetwork.timeconstant  thermal_mass=[3, 25] J/K  thermal_mass_Cauer=[3, 10, 25] J/K  thermal_mass_Foster=[.001, .005, .05, .5] J/K  thermal_time_constant=[.1, 5] s  thermal_time_constant_Cauer=[.1, 1, 5] s  thermal_time_constant_Foster=[7e-05, .0007, .01, .08] s  thermal_mass_initial_temperatures=[25, 25] degC  thermal_mass_initial_temperatures_Cauer=[25, 25, 25] degC  junction_thermal_mass=0.1 J/K  Tvec_initial_Foster=[25, 25, 25, 25] degC  RthDiode=[.03, .2] K/W  RthCauerDiode=[.03, .1, .2] K/W  RthFosterDiode=[.03, .2] K/W  thermalMassDiode=[3, 25] J/K  thermalMassCauerDiode=[3, 10, 25] J/K  thermalMassFosterDiode=[33, 50] J/K  thermalTauDiode=[.1, 5] s  thermalTauCauerDiode=[.1, 1, 5] s  thermalTauFosterDiode=[1, 10] s  thermalMassInitTempDiode=[25, 25] degC  thermalMassInitTempCauerDiode=[25, 25, 25] degC  junctionthermalMassDiode=0.1 J/K  TVecInitialFosterDiode=[25, 25, 25, 25] degC  no_thermal_network=ee.enum.enable.no  mosfet_junction_temperature_specify=off  mosfet_junction_temperature_priority=None  mosfet_junction_temperature=25 degC  mosfet_junction_temperature_nominal_specify=off  mosfet_junction_temperature_nominal_value=1  mosfet_junction_temperature_nominal_unit=degC  diode_junction_temperature_specify=off  diode_junction_temperature_priority=None  diode_junction_temperature=25 degC  diode_junction_temperature_nominal_specify=off  diode_junction_temperature_nominal_value=1  diode_junction_temperature_nominal_unit=degC  Qj_specify=off  Qj_priority=None  Qj=0 W  Qj_nominal_specify=off  Qj_nominal_value=1  Qj_nominal_unit=W  accumulatedSwitchingLosses_specify=off  accumulatedSwitchingLosses_priority=None  accumulatedSwitchingLosses=0 J
  Output current sensor : fl_lib/Electrical/Electrical Sensors/Current Sensor
  PS-S I : nesl_utility/PS-Simulink Converter  PhysicalDomain=network_engine_domain  SubClassName=ps_output  LeftPortType=input  RightPortType=output  PseudoPeriodic=off  Frequencies=[]  VectorFormat=inherit  Unit=inherit  AffineConversion=off
  PS-S Vsw : nesl_utility/PS-Simulink Converter  PhysicalDomain=network_engine_domain  SubClassName=ps_output  LeftPortType=input  RightPortType=output  PseudoPeriodic=off  Frequencies=[]  VectorFormat=inherit  Unit=inherit  AffineConversion=off
  Switch-node voltage sensor : fl_lib/Electrical/Electrical Sensors/Voltage Sensor
  DC+ : PMIOPort  Side=Left
  DC- : PMIOPort  Port=2  Side=Left
  OUT : PMIOPort  Port=3  Side=Right
  I_out : Outport
  V_sw : Outport  Port=2
  wires:
  Vgs_H/1 -> Gate driver H/1
  Vgs_L/1 -> Gate driver L/1
  PS-S I/1 -> I_out/1
  PS-S Vsw/1 -> V_sw/1
  connections:
  Gate driver H/RConn1 -- High-side 4x IRFP90N20D/LConn1
  Gate driver L/RConn1 -- Low-side 4x IRFP90N20D/LConn1
  DC+/RConn1 -- High-side 4x IRFP90N20D/RConn1
  Output current sensor/LConn1 -- High-side 4x IRFP90N20D/RConn2 -- Low-side 4x IRFP90N20D/RConn1 -- Switch-node voltage sensor/LConn1
  DC-/RConn1 -- Switch-node voltage sensor/RConn2 -- Low-side 4x IRFP90N20D/RConn2
  Output current sensor/RConn2 -- OUT/RConn1
  Output current sensor/RConn1 -- PS-S I/LConn1
  Switch-node voltage sensor/RConn1 -- PS-S Vsw/LConn1
